simulink model "r2_b8a4x128f_4gbe"  (R2012b)
settings: Solver=VariableStepDiscrete  SolverMode=SingleTasking  StartTime=0.0  StopTime=1  RelTol=1e-3
undefined symbols (not defined in the file): fft_stages, n_ants, n_bits_xengs
libraries: xbsIndex_r4 x21845, casper_library_misc x157, xbsReplacements_r4 x24, casper_library_communications x8, casper_library_delays x8, xps_library x5
(part 77 of 182)

== system r2_b8a4x128f_4gbe/sys2/bf/fbf ==
  note: beam filtering
  note: requanitse
  note: accumulate
  note: create visibilities
  note: combine data from different antennas into beams
  note: beam steering
  note: antenna beam weights
  note: split polarisations and
      | duplicate for multiple beams
  note: TODO
  note: TODO
  note: control interface
  note: TODO
  synci : Inport
  di : Inport  Port=2
  deni : Inport  Port=3
  badi : Inport  Port=4
  timei : Inport  Port=5
  misci : Inport  Port=6
  ld_antenna : Inport  Port=7
  ld_stream : Inport  Port=8
  ld_wr_en : Inport  Port=9
  Assert : xbsIndex_r4/Assert  assert_type=on  type_source=Explicitly  gui_display_data_type=Boolean  arith_type=Boolean  n_bits=16  bin_pt=14  preci_type=Single  exp_width=8  frac_width=24  assert_rate=off  rate_source=Explicitly  period=1  output_port=on  block_type=assert
  Assert1 : xbsIndex_r4/Assert  assert_type=on  type_source=Explicitly  gui_display_data_type=Boolean  arith_type=Boolean  n_bits=16  bin_pt=14  preci_type=Single  exp_width=8  frac_width=24  assert_rate=off  rate_source=Explicitly  period=1  output_port=on  block_type=assert
  Assert2 : xbsIndex_r4/Assert  assert_type=on  type_source=Explicitly  gui_display_data_type=Boolean  arith_type=Boolean  n_bits=16  bin_pt=14  preci_type=Single  exp_width=8  frac_width=24  assert_rate=off  rate_source=Explicitly  period=1  output_port=on  block_type=assert
  Assert3 : xbsIndex_r4/Assert  assert_type=on  type_source=Explicitly  gui_display_data_type=Fixed-point  arith_type=Unsigned  n_bits=n_bits_in*2*2^polarisation_bits  bin_pt=0  preci_type=Single  exp_width=8  frac_width=24  assert_rate=off  rate_source=Explicitly  period=1  output_port=on  block_type=assert
  Assert4 : xbsIndex_r4/Assert  assert_type=on  type_source=Explicitly  gui_display_data_type=Fixed-point  arith_type=Unsigned  n_bits=timestamp_bits  bin_pt=0  preci_type=Single  exp_width=8  frac_width=24  assert_rate=off  rate_source=Explicitly  period=1  output_port=on  block_type=assert
  Assert6 : xbsIndex_r4/Assert  assert_type=on  type_source=Explicitly  gui_display_data_type=Fixed-point  arith_type=Unsigned  n_bits=ant_bits  bin_pt=0  preci_type=Single  exp_width=8  frac_width=24  assert_rate=off  rate_source=Explicitly  period=1  output_port=on  block_type=assert
  Assert7 : xbsIndex_r4/Assert  assert_type=on  type_source=Explicitly  gui_display_data_type=Fixed-point  arith_type=Unsigned  n_bits=polarisation_bits+beam_bits  bin_pt=0  preci_type=Single  exp_width=8  frac_width=24  assert_rate=off  rate_source=Explicitly  period=1  output_port=on  block_type=assert
  Assert9 : xbsIndex_r4/Assert  assert_type=on  type_source=Explicitly  gui_display_data_type=Boolean  arith_type=Boolean  n_bits=8  bin_pt=0  preci_type=Single  exp_width=8  frac_width=24  assert_rate=off  rate_source=Explicitly  period=1  output_port=on  block_type=assert
  Concat : xbsIndex_r4/Concat  num_inputs=2  dbl_ovrd=off  block_type=concat
  Concat1 : xbsIndex_r4/Concat  num_inputs=3  dbl_ovrd=off  block_type=concat
  Concat2 : xbsIndex_r4/Concat  num_inputs=2  dbl_ovrd=off  block_type=concat
  Concat3 : xbsIndex_r4/Concat  num_inputs=2  dbl_ovrd=off  block_type=concat
  Constant4 : xbsIndex_r4/Constant  const=0  gui_display_data_type=Fixed-point  arith_type=Unsigned  n_bits=freq_bits-beng_bits  bin_pt=0  preci_type=Single  exp_width=8  frac_width=24  explicit_period=on  period=1  equ=P=C  opselect=C  inp2=PCIN>>17  opr=+  inp1=P  carry=CIN  dbl_ovrd=off  block_type=constant
      settings: block_version=11.4
  Convert4 : xbsIndex_r4/Convert  gui_display_data_type=Fixed-point  arith_type=Unsigned  n_bits=1  bin_pt=0  float_type=Single  exp_bits=8  fraction_bits=24  quantization=Truncate  overflow=Wrap  en=off  latency=0  dbl_ovrd=off  pipeline=off  block_type=convert
  Delay{1..3,7} (4 alike) : xbsIndex_r4/Delay  rst=off  infoeditControl=Selection of Reset will increase slice count due to use of real FFs and instead of SRLs  en=off  latency=1  dbl_ovrd=off  reg_retiming=on  block_type=delay
  Gateway Out{,1..18} (19 alike) : xbsIndex_r4/Gateway Out  inherit_from_input=off  hdl_port=off  timing_constraint=None  locs_specified=off  LOCs={}  UseAsDAC=off  DACChannel='1'  block_type=gatewayout
      settings: infoedit="Gateway out block.  Converts Xilinx fixed point inputs into ouputs of type Simulink integer, double, or fixed point.<br><br>Hardware notes:  In hardware these blocks become top level output ports or are discarded, depending on how they are configured."  block_version=11.4
  Logical{,1..3} (4 alike) : xbsIndex_r4/Logical  logical_function=AND  inputs=2  en=off  latency=1  precision=Full  arith_type=Unsigned  n_bits=16  bin_pt=0  align_bp=on  dbl_ovrd=off  block_type=logical
  Reinterpret : xbsIndex_r4/Reinterpret  force_arith_type=on  arith_type="Signed  (2's comp)"  force_bin_pt=on  bin_pt=bin_pt_norm  block_type=reinterpret
      settings: infoedit="Changes signal type without altering the binary representation.   You can changed the signal between signed and unsigned, and relocate the binary point.<br><br>Hardware notes: In hardware this block costs nothing.<br><br>Example:  Suppose the input is 6 bits wide, signed, with 2 fractional bits, and the output is forced to unsigned with 0 fractional bits.  Then an input of -2.0 (1110.00 in binary 2's complement) becomes an output of 56 (111000 in binary)."
  Reinterpret1 : xbsIndex_r4/Reinterpret  force_arith_type=on  arith_type="Signed  (2's comp)"  force_bin_pt=on  bin_pt=bin_pt_norm  block_type=reinterpret
      settings: infoedit="Changes signal type without altering the binary representation.   You can changed the signal between signed and unsigned, and relocate the binary point.<br><br>Hardware notes: In hardware this block costs nothing.<br><br>Example:  Suppose the input is 6 bits wide, signed, with 2 fractional bits, and the output is forced to unsigned with 0 fractional bits.  Then an input of -2.0 (1110.00 in binary 2's complement) becomes an output of 56 (111000 in binary)."
  Reinterpret10 : xbsIndex_r4/Reinterpret  force_arith_type=on  arith_type=Unsigned  force_bin_pt=on  bin_pt=0  block_type=reinterpret
  Reinterpret11 : xbsIndex_r4/Reinterpret  force_arith_type=on  arith_type=Unsigned  force_bin_pt=on  bin_pt=0  block_type=reinterpret
  Reinterpret{2..3,6..9} (6 alike) : xbsIndex_r4/Reinterpret  force_arith_type=on  arith_type="Signed  (2's comp)"  force_bin_pt=on  bin_pt=0  block_type=reinterpret
      settings: infoedit="Changes signal type without altering the binary representation.   You can changed the signal between signed and unsigned, and relocate the binary point.<br><br>Hardware notes: In hardware this block costs nothing.<br><br>Example:  Suppose the input is 6 bits wide, signed, with 2 fractional bits, and the output is forced to unsigned with 0 fractional bits.  Then an input of -2.0 (1110.00 in binary 2's complement) becomes an output of 56 (111000 in binary)."
  Reinterpret4 : xbsIndex_r4/Reinterpret  force_arith_type=on  arith_type="Signed  (2's comp)"  force_bin_pt=on  bin_pt=bin_pt_out  block_type=reinterpret
      settings: infoedit="Changes signal type without altering the binary representation.   You can changed the signal between signed and unsigned, and relocate the binary point.<br><br>Hardware notes: In hardware this block costs nothing.<br><br>Example:  Suppose the input is 6 bits wide, signed, with 2 fractional bits, and the output is forced to unsigned with 0 fractional bits.  Then an input of -2.0 (1110.00 in binary 2's complement) becomes an output of 56 (111000 in binary)."
  Reinterpret5 : xbsIndex_r4/Reinterpret  force_arith_type=on  arith_type="Signed  (2's comp)"  force_bin_pt=on  bin_pt=bin_pt_out  block_type=reinterpret
      settings: infoedit="Changes signal type without altering the binary representation.   You can changed the signal between signed and unsigned, and relocate the binary point.<br><br>Hardware notes: In hardware this block costs nothing.<br><br>Example:  Suppose the input is 6 bits wide, signed, with 2 fractional bits, and the output is forced to unsigned with 0 fractional bits.  Then an input of -2.0 (1110.00 in binary 2's complement) becomes an output of 56 (111000 in binary)."
  Scope : Scope  NumInputPorts=5
      settings: YMin=0~-15~-15~0~10  YMax=1~12.5~12.5~1~11  SaveName=ScopeData2
  Scope1 : Scope  NumInputPorts=4
      settings: YMin=0~-1~0~-5  YMax=1~1~1~5  SaveName=ScopeData5
  Scope2 : Scope  NumInputPorts=4
      settings: YMin=0.1~-1~0~-5  YMax=1~0.5~1~5  SaveName=ScopeData14
  Scope3 : Scope  NumInputPorts=6
      settings: YMin=-1~3~3~3~3~-1  YMax=1~5~5~5~5~1  SaveName=ScopeData8
  Slice : xbsIndex_r4/Slice  nbits=n_bits_combine  boolean_output=off  mode=Lower Bit Location + Width  bit1=0  base1=MSB of Input  bit0=0  base0=LSB of Input  dbl_ovrd=off  block_type=slice
  Slice1 : xbsIndex_r4/Slice  nbits=n_bits_combine  boolean_output=off  mode=Lower Bit Location + Width  bit1=0  base1=MSB of Input  bit0=n_bits_combine  base0=LSB of Input  dbl_ovrd=off  block_type=slice
  Slice2 : xbsIndex_r4/Slice  nbits=n_bits_out  boolean_output=off  mode=Lower Bit Location + Width  bit1=0  base1=MSB of Input  bit0=0  base0=LSB of Input  dbl_ovrd=off  block_type=slice
  Slice3 : xbsIndex_r4/Slice  nbits=n_bits_out  boolean_output=off  mode=Lower Bit Location + Width  bit1=0  base1=MSB of Input  bit0=n_bits_out  base0=LSB of Input  dbl_ovrd=off  block_type=slice
  Slice4 : xbsIndex_r4/Slice  nbits=n_bits_out  boolean_output=off  mode=Lower Bit Location + Width  bit1=0  base1=MSB of Input  bit0=0  base0=LSB of Input  dbl_ovrd=off  block_type=slice
  Slice5 : xbsIndex_r4/Slice  nbits=n_bits_out  boolean_output=off  mode=Lower Bit Location + Width  bit1=0  base1=MSB of Input  bit0=n_bits_out  base0=LSB of Input  dbl_ovrd=off  block_type=slice
  Slice7 : xbsIndex_r4/Slice  nbits=1  boolean_output=on  mode=Lower Bit Location + Width  bit1=0  base1=MSB of Input  bit0=0  base0=LSB of Input  dbl_ovrd=off  block_type=slice
  apply_beam_weights : Subsystem  mask{vec_bits=ant_bits, stream_bits=polarisation_bits+beam_bits, stack_bits=(freq_bits-beng_bits)+stack_bits, type_in=1, n_bits_in=n_bits_in, bin_pt_in=bin_pt_in, complex_in=on, type_coeff=1, n_bits_coeff=n_bits_norm, bin_pt_coeff=bin_pt_norm, complex_coeff=off, mult_latency=mult_latency, n_bits_out=n_bits_in+n_bits_norm+1, bin_pt_out=bin_pt_in+bin_pt_norm, type_out=1, quantization=0, overflow=0, init_val=1}
      mask prompts: vec_bits "vector length (2^?)"; stream_bits "streams (2^?)"; stack_bits "stack factor (2^?)"; type_in "input type (Unsigned=0, Signed=1)"; n_bits_in "bit width in"; bin_pt_in "binary point in"; complex_in "complex input"; type_coeff "coefficient type (Unsigned=0, Signed=1)"; n_bits_coeff "coefficient bit width"; bin_pt_coeff "coefficient binary point"; complex_coeff "complex coefficients"; mult_latency "multiplier latency"; n_bits_out "output bit width"; bin_pt_out "output binary point"; type_out "output type (Unsigned=0, Signed=1)"; quantization "quantization strategy (Truncate=0, Round  (unbiased: +/- Inf)=1)"; overflow "overflow strategy (Wrap=0, Saturate=1, Flag as error=2)"; init_val "initial value"
      mask init: same as r2_b8a4x128f_4gbe/sys0/bf/fbf/apply_beam_weights
  bad_slc : xbsIndex_r4/Slice  nbits=1  boolean_output=on  mode=Upper Bit Location + Width  bit1=0  base1=MSB of Input  bit0=0  base0=LSB of Input  dbl_ovrd=off  block_type=slice
  bus_expand : Subsystem  AncestorBlock=casper_library_flow_control/bus_expand  mask(bus_expand){mode=divisions of equal size, outputNum=4, outputWidth=4, outputBinaryPt=3, outputArithmeticType=1, show_format=off, outputToWorkspace=off, variablePrefix=out, outputToModelAsWell=on}
      mask prompts: outputNum "Number of outputs:"; outputWidth "Output width:"; outputBinaryPt "Output binary point position:"; outputArithmeticType "Output arithmetic type (ufix=0, fix=1, bool=2):"; show_format "Print format string?"; outputToWorkspace "Output to workspace?"; variablePrefix "Variable name prefix:"; outputToModelAsWell "Output to model as well?"
      mask help:
      | Expands a 'bus' made using a bus_create or Xilinx
      | concat block.
      | The input will be divided into the specified number
      | of outputs with the specified arithmetic types.
      | Divisions are made from most significant bit.
      mask init: same as r2_b8a4x128f_4gbe/bus_expand
      settings: AttributesFormatString=4 outputs
      mask TypeOptions mode: divisions of equal size | divisions of arbitrary size
      mask Callback mode: bus_expand_callback();
      mask Callback outputWidth: bus_expand_callback();
      mask Callback outputToWorkspace: bus_expand_callback();
  combine : Subsystem  mask{freq_bits=freq_bits-beng_bits, ant_bits=ant_bits, stack_bits=stack_bits, stream_bits=beam_bits+polarisation_bits, n_bits_in=n_bits_in+n_bits_norm+1, bin_pt_in=bin_pt_in+bin_pt_norm, timestamp_bits=timestamp_bits, n_bits_accum=n_bits_combine, bram_latency=bram_latency, add_latency=add_latency}
      mask prompts: freq_bits "frequencies (2^?)"; ant_bits "antennas (2^?)"; stack_bits "stacking factor (2^?)"; stream_bits "input streams (2^?)"; n_bits_in "data bits in"; bin_pt_in "binary point in"; timestamp_bits "timestamp bits"; n_bits_accum "accumulator bits"; bram_latency "bram latency"; add_latency "add latency"
  duplicate : Subsystem  mask{ant_bits=ant_bits, freq_bits=freq_bits-beng_bits, stack_bits=stack_bits, beam_bits=beam_bits, polarisation_bits=polarisation_bits, n_bits_in=n_bits_in}
      mask prompts: ant_bits "antennas (2^?)"; freq_bits "frequencies (2^?)"; stack_bits "stacking factor (2^?)"; beam_bits "beams (2^?)"; polarisation_bits "polarisations (2^?)"; n_bits_in "data bits in"
      mask init:
      | set_param([gcb,'/beam_replicate'], ...
      |     'replication', '2^beam_bits');
      | set_param([gcb,'/pol_replicate'], ...
      |     'replication', '2^polarisation_bits');
  filter : Subsystem  mask{stream_bits=beam_bits+polarisation_bits, vec_bits=freq_bits-beng_bits, stack_bits=stack_bits, output_enabled=off}
      mask prompts: stream_bits "streams (2^?)"; vec_bits "vector length (2^?)"; stack_bits "stack factor (2^?)"; output_enabled "output enabled by default?"
      mask init: same as r2_b8a4x128f_4gbe/sys0/bf/fbf/filter
  ld_freq5 : xbsIndex_r4/Slice  nbits=1  boolean_output=off  mode=Two Bit Locations  bit1=-(timestamp_bits+1)  base1=MSB of Input  bit0=0  base0=LSB of Input  dbl_ovrd=off  block_type=slice
  misco_slc : xbsIndex_r4/Slice  nbits=1  boolean_output=off  mode=Two Bit Locations  bit1=-timestamp_bits  base1=MSB of Input  bit0=0  base0=LSB of Input  dbl_ovrd=off  block_type=slice
  pipeline1 : Subsystem  AncestorBlock=casper_library_delays/pipeline  mask(pipeline){latency=2}
      mask help:
      | An explicitly laid-out delay line to avoid mapping to SRL16s
      | for use in pipelining to help achieve timing closure.
      mask init:
      | pipeline_init(gcb,'latency',latency);
      settings: AttributesFormatString=Latency = %<latency>
      mask Display:
      | port_label('input', 1, 'd');
      | port_label('output', 1, 'q');
      | disp(['Z^-', num2str(latency)]);
  pipeline10 : Subsystem  AncestorBlock=casper_library_delays/pipeline  mask(pipeline){latency=2}
      mask help:
      | An explicitly laid-out delay line to avoid mapping to SRL16s
      | for use in pipelining to help achieve timing closure.
      mask init:
      | pipeline_init(gcb,'latency',latency);
      settings: AttributesFormatString=Latency = %<latency>
      mask Display:
      | port_label('input', 1, 'd');
      | port_label('output', 1, 'q');
      | disp(['Z^-', num2str(latency)]);
  pipeline11 : Subsystem  AncestorBlock=casper_library_delays/pipeline  mask(pipeline){latency=2}
      mask help:
      | An explicitly laid-out delay line to avoid mapping to SRL16s
      | for use in pipelining to help achieve timing closure.
      mask init:
      | pipeline_init(gcb,'latency',latency);
      settings: AttributesFormatString=Latency = %<latency>
      mask Display:
      | port_label('input', 1, 'd');
      | port_label('output', 1, 'q');
      | disp(['Z^-', num2str(latency)]);
  pipeline12 : Subsystem  AncestorBlock=casper_library_delays/pipeline  mask(pipeline){latency=2}
      mask help:
      | An explicitly laid-out delay line to avoid mapping to SRL16s
      | for use in pipelining to help achieve timing closure.
      mask init:
      | pipeline_init(gcb,'latency',latency);
      settings: AttributesFormatString=Latency = %<latency>
      mask Display:
      | port_label('input', 1, 'd');
      | port_label('output', 1, 'q');
      | disp(['Z^-', num2str(latency)]);
  pipeline13 : Subsystem  AncestorBlock=casper_library_delays/pipeline  mask(pipeline){latency=2}
      mask help:
      | An explicitly laid-out delay line to avoid mapping to SRL16s
      | for use in pipelining to help achieve timing closure.
      mask init:
      | pipeline_init(gcb,'latency',latency);
      settings: AttributesFormatString=Latency = %<latency>
      mask Display:
      | port_label('input', 1, 'd');
      | port_label('output', 1, 'q');
      | disp(['Z^-', num2str(latency)]);
  pipeline14 : Subsystem  AncestorBlock=casper_library_delays/pipeline  mask(pipeline){latency=2}
      mask help:
      | An explicitly laid-out delay line to avoid mapping to SRL16s
      | for use in pipelining to help achieve timing closure.
      mask init:
      | pipeline_init(gcb,'latency',latency);
      settings: AttributesFormatString=Latency = %<latency>
      mask Display:
      | port_label('input', 1, 'd');
      | port_label('output', 1, 'q');
      | disp(['Z^-', num2str(latency)]);
  pipeline15 : Subsystem  AncestorBlock=casper_library_delays/pipeline  mask(pipeline){latency=2}
      mask help:
      | An explicitly laid-out delay line to avoid mapping to SRL16s
      | for use in pipelining to help achieve timing closure.
      mask init:
      | pipeline_init(gcb,'latency',latency);
      settings: AttributesFormatString=Latency = %<latency>
      mask Display:
      | port_label('input', 1, 'd');
      | port_label('output', 1, 'q');
      | disp(['Z^-', num2str(latency)]);
  pipeline16 : Subsystem  AncestorBlock=casper_library_delays/pipeline  mask(pipeline){latency=2}
      mask help:
      | An explicitly laid-out delay line to avoid mapping to SRL16s
      | for use in pipelining to help achieve timing closure.
      mask init:
      | pipeline_init(gcb,'latency',latency);
      settings: AttributesFormatString=Latency = %<latency>
      mask Display:
      | port_label('input', 1, 'd');
      | port_label('output', 1, 'q');
      | disp(['Z^-', num2str(latency)]);
  pipeline2 : Subsystem  AncestorBlock=casper_library_delays/pipeline  mask(pipeline){latency=2}
      mask help:
      | An explicitly laid-out delay line to avoid mapping to SRL16s
      | for use in pipelining to help achieve timing closure.
      mask init:
      | pipeline_init(gcb,'latency',latency);
      settings: AttributesFormatString=Latency = %<latency>
      mask Display:
      | port_label('input', 1, 'd');
      | port_label('output', 1, 'q');
      | disp(['Z^-', num2str(latency)]);
  pipeline3 : Subsystem  AncestorBlock=casper_library_delays/pipeline  mask(pipeline){latency=2}
      mask help:
      | An explicitly laid-out delay line to avoid mapping to SRL16s
      | for use in pipelining to help achieve timing closure.
      mask init:
      | pipeline_init(gcb,'latency',latency);
      settings: AttributesFormatString=Latency = %<latency>
      mask Display:
      | port_label('input', 1, 'd');
      | port_label('output', 1, 'q');
      | disp(['Z^-', num2str(latency)]);
  pipeline4 : Subsystem  AncestorBlock=casper_library_delays/pipeline  mask(pipeline){latency=2}
      mask help:
      | An explicitly laid-out delay line to avoid mapping to SRL16s
      | for use in pipelining to help achieve timing closure.
      mask init:
      | pipeline_init(gcb,'latency',latency);
      settings: AttributesFormatString=Latency = %<latency>
      mask Display:
      | port_label('input', 1, 'd');
      | port_label('output', 1, 'q');
      | disp(['Z^-', num2str(latency)]);
  pipeline5 : Subsystem  AncestorBlock=casper_library_delays/pipeline  mask(pipeline){latency=2}
      mask help:
      | An explicitly laid-out delay line to avoid mapping to SRL16s
      | for use in pipelining to help achieve timing closure.
      mask init:
      | pipeline_init(gcb,'latency',latency);
      settings: AttributesFormatString=Latency = %<latency>
      mask Display:
      | port_label('input', 1, 'd');
      | port_label('output', 1, 'q');
      | disp(['Z^-', num2str(latency)]);
  pipeline6 : Subsystem  AncestorBlock=casper_library_delays/pipeline  mask(pipeline){latency=2}
      mask help:
      | An explicitly laid-out delay line to avoid mapping to SRL16s
      | for use in pipelining to help achieve timing closure.
      mask init:
      | pipeline_init(gcb,'latency',latency);
      settings: AttributesFormatString=Latency = %<latency>
      mask Display:
      | port_label('input', 1, 'd');
      | port_label('output', 1, 'q');
      | disp(['Z^-', num2str(latency)]);
  pipeline7 : Subsystem  AncestorBlock=casper_library_delays/pipeline  mask(pipeline){latency=2}
      mask help:
      | An explicitly laid-out delay line to avoid mapping to SRL16s
      | for use in pipelining to help achieve timing closure.
      mask init:
      | pipeline_init(gcb,'latency',latency);
      settings: AttributesFormatString=Latency = %<latency>
      mask Display:
      | port_label('input', 1, 'd');
      | port_label('output', 1, 'q');
      | disp(['Z^-', num2str(latency)]);
  pipeline8 : Subsystem  AncestorBlock=casper_library_delays/pipeline  mask(pipeline){latency=2}
      mask help:
      | An explicitly laid-out delay line to avoid mapping to SRL16s
      | for use in pipelining to help achieve timing closure.
      mask init:
      | pipeline_init(gcb,'latency',latency);
      settings: AttributesFormatString=Latency = %<latency>
      mask Display:
      | port_label('input', 1, 'd');
      | port_label('output', 1, 'q');
      | disp(['Z^-', num2str(latency)]);
  pipeline9 : Subsystem  AncestorBlock=casper_library_delays/pipeline  mask(pipeline){latency=2}
      mask help:
      | An explicitly laid-out delay line to avoid mapping to SRL16s
      | for use in pipelining to help achieve timing closure.
      mask init:
      | pipeline_init(gcb,'latency',latency);
      settings: AttributesFormatString=Latency = %<latency>
      mask Display:
      | port_label('input', 1, 'd');
      | port_label('output', 1, 'q');
      | disp(['Z^-', num2str(latency)]);
  requantise : Subsystem  mask{vec_bits=freq_bits-beng_bits, stream_bits=polarisation_bits+beam_bits, stack_bits=stack_bits, type_in=1, n_bits_in=n_bits_combine, bin_pt_in=bin_pt_in+bin_pt_norm, complex_in=on, type_coeff=1, n_bits_coeff=n_bits_requant, bin_pt_coeff=bin_pt_requant, complex_coeff=off, mult_latency=mult_latency, conv_latency=conv_latency, n_bits_out=n_bits_out, bin_pt_out=bin_pt_out, type_out=1, quantization=1, overflow=1, init_val=1}
      mask prompts: vec_bits "vector length (2^?)"; stream_bits "streams (2^?)"; stack_bits "stack factor (2^?)"; type_in "input type (Unsigned=0, Signed=1)"; n_bits_in "bit width in"; bin_pt_in "binary point in"; complex_in "complex input"; type_coeff "coefficient type (Unsigned=0, Signed=1)"; n_bits_coeff "coefficient bit width"; bin_pt_coeff "coefficient binary point"; complex_coeff "complex coefficients"; mult_latency "multiplier latency"; conv_latency "convert latency"; n_bits_out "output bit width"; bin_pt_out "output binary point"; type_out "output type (Unsigned=0, Signed=1)"; quantization "quantization strategy (Truncate=0, Round  (unbiased: +/- Inf)=1)"; overflow "overflow strategy (Wrap=0, Saturate=1, Flag as error=2)"; init_val "initial value"
      mask init: same as r2_b8a4x128f_4gbe/sys0/bf/fbf/requantise
  sync_gen : Subsystem
  time_slc : xbsIndex_r4/Slice  nbits=timestamp_bits  boolean_output=off  mode=Upper Bit Location + Width  bit1=-1  base1=MSB of Input  bit0=0  base0=LSB of Input  dbl_ovrd=off  block_type=slice
  timeo_slc : xbsIndex_r4/Slice  nbits=timestamp_bits  boolean_output=off  mode=Upper Bit Location + Width  bit1=0  base1=MSB of Input  bit0=0  base0=LSB of Input  dbl_ovrd=off  block_type=slice
  synco : Outport
  do : Outport  Port=2
  deno : Outport  Port=3
  timeo : Outport  Port=4
  misco : Outport  Port=5
  bw_value_out : Outport  Port=6
  quant_value_out : Outport  Port=7
  filter_value_out : Outport  Port=8
  wires:
  sync_gen/3(do) -> duplicate/3(di)
  sync_gen/6(misco) -> duplicate/6(misci)
  sync_gen/5(timeo) -> duplicate/5(timei)
  sync_gen/2(dvalid) -> duplicate/2(eni)
  sync_gen/1(synco) -> duplicate/1(synci)
  sync_gen/4(bado) -> duplicate/4(badi)
  misci/1 -> sync_gen/6(misci)
  Assert4/1 -> sync_gen/5(timei)
  Assert2/1 -> sync_gen/4(badi)
  Assert3/1 -> sync_gen/3(di)
  Assert/1 -> sync_gen/1(synci)
  Assert1/1 -> sync_gen/2(en)
  Assert9/1 -> [control_en]
  ld_wr_en/1 -> Assert9/1
  Assert7/1 -> [stream]
  ld_stream/1 -> Assert7/1
  Assert6/1 -> [antenna]
  ld_antenna/1 -> Assert6/1
  Gateway Out5/1 -> Scope1/4
  Gateway Out4/1 -> Scope1/3
  Gateway Out3/1 -> Scope1/2
  Gateway Out18/1 -> Scope1/1
  [requantise_synco] -> Gateway Out18/1
  filter/1(synco) -> [filter_synco], synco/1
  requantise/1(synco) -> pipeline4/1(d), [requantise_synco]
  [requantise_val_out] -> quant_value_out/1
  [filter_val_out] -> filter_value_out/1
  requantise/5(valo) -> [requantise_val_out]
  filter/5(valo) -> [filter_val_out]
  [bw_val_out] -> bw_value_out/1
  apply_beam_weights/5(valo) -> [bw_val_out]
  apply_beam_weights/4(misco) -> pipeline11/1(d)
  [filter_synco] -> Gateway Out17/1
  Gateway Out9/1 -> Scope2/4
  Gateway Out8/1 -> Scope2/3
  Gateway Out7/1 -> Scope2/2
  Gateway Out17/1 -> Scope2/1
  Gateway Out14/1 -> Scope3/6
  Gateway Out13/1 -> Scope3/5
  Gateway Out12/1 -> Scope3/4
  Gateway Out11/1 -> Scope3/3
  Gateway Out10/1 -> Scope3/2
  Gateway Out16/1 -> Scope3/1
  [gen_sync] -> Gateway Out16/1
  Gateway Out6/1 -> Scope/5
  Gateway Out2/1 -> Scope/4
  Gateway Out1/1 -> Scope/3
  Gateway Out/1 -> Scope/2
  Gateway Out15/1 -> Scope/1
  [combine_sync] -> Gateway Out15/1
  filter/3(eno) -> [filter_eno], deno/1
  filter/2(do) -> [filter_dout], do/1
  requantise/4(misco) -> pipeline7/1(d)
  requantise/3(eno) -> pipeline6/1(d), [requantise_eno]
  requantise/2(dout) -> pipeline5/1(d), [requantise_dout]
  combine/1(synco) -> pipeline15/1(d), [combine_sync]
  apply_beam_weights/1(synco) -> pipeline8/1(d)
  filter/4(misco) -> misco_slc/1, timeo_slc/1
  [gen_do] -> bus_expand/1(bus_in)
  bus_expand/4(lsb_out1) -> Reinterpret9/1
  bus_expand/3(out2) -> Reinterpret8/1
  [gen_eno] -> Gateway Out14/1
  Reinterpret9/1 -> Gateway Out13/1
  Reinterpret8/1 -> Gateway Out12/1
  Reinterpret7/1 -> Gateway Out11/1
  Reinterpret6/1 -> Gateway Out10/1
  bus_expand/2(out3) -> Reinterpret7/1
  bus_expand/1(msb_out4) -> Reinterpret6/1
  Convert4/1 -> Slice7/1
  [bf_value_dupl] -> Delay3/1
  Reinterpret5/1 -> Gateway Out8/1
  Reinterpret4/1 -> Gateway Out7/1
  [filter_eno] -> Gateway Out9/1
  [filter_dout] -> Slice4/1, Slice5/1
  Slice4/1 -> Reinterpret5/1
  Slice5/1 -> Reinterpret4/1
  [stream] -> filter/5(stream)
  [combine_time] -> Gateway Out6/1
  Concat3/1 -> pipeline3/1(d)
  combine/5(misco) -> Concat3/2
  combine/4(timeo) -> [combine_time], Concat3/1
  time_slc/1 -> combine/5(timei)
  duplicate/5(timeo) -> Concat1/2
  duplicate/4(bado) -> Concat1/1
  duplicate/3(eno) -> pipeline14/1(d), [gen_eno]
  misco_slc/1 -> misco/1
  timeo_slc/1 -> timeo/1
  Reinterpret3/1 -> Gateway Out4/1
  Reinterpret2/1 -> Gateway Out3/1
  [requantise_eno] -> Gateway Out5/1
  [requantise_dout] -> Slice3/1, Slice2/1
  Slice2/1 -> Reinterpret3/1
  Slice3/1 -> Reinterpret2/1
  Reinterpret1/1 -> Gateway Out1/1
  Reinterpret/1 -> Gateway Out/1
  [combine_eno] -> Gateway Out2/1
  [combine_sum] -> Slice/1, Slice1/1
  Slice/1 -> Reinterpret1/1
  Slice1/1 -> Reinterpret/1
  apply_beam_weights/3(eno) -> pipeline10/1(d)
  apply_beam_weights/2(dout) -> pipeline9/1(d)
  combine/3(eno) -> pipeline2/1(d), [combine_eno]
  combine/2(sum) -> pipeline1/1(d), [combine_sum]
  Delay7/1 -> Reinterpret11/1
  duplicate/6(misco) -> Concat1/3
  Logical1/1 -> apply_beam_weights/7(we)
  Delay2/1 -> Reinterpret10/1
  Concat/1 -> apply_beam_weights/5(index)
  timei/1 -> Assert4/1
  ld_freq5/1 -> combine/6(misci)
  bad_slc/1 -> combine/4(bad)
  Concat1/1 -> pipeline16/1(d)
  duplicate/2(do) -> pipeline13/1(d), [gen_do]
  duplicate/1(synco) -> pipeline12/1(d), [gen_sync]
  badi/1 -> Assert2/1
  di/1 -> Assert3/1
  deni/1 -> Assert1/1
  synci/1 -> Assert/1
  [antenna] -> Concat/1
  [stream] -> Concat/2
  [frequency] -> Concat2/1
  [stream] -> Concat2/2
  Concat2/1 -> requantise/5(index)
  Constant4/1 -> [frequency]
  Delay1/1 -> filter/6(vali)
  Slice7/1 -> duplicate/8(sim_type)
  Reinterpret10/1 -> apply_beam_weights/6(vali)
  Reinterpret11/1 -> requantise/6(vali)
  Delay3/1 -> Convert4/1
  [bf_value_filt] -> Delay1/1
  [bf_value_bw] -> Delay2/1
  [bf_value_quant] -> Delay7/1
  Logical2/1 -> requantise/7(we)
  Logical3/1 -> filter/7(ld)
  [control_en] -> Logical/2
  [bf_valctrl_dupl] -> Logical/1
  Logical/1 -> duplicate/7(sim_ld)
  [control_en] -> Logical1/2
  [bf_valctrl_bw] -> Logical1/1
  [control_en] -> Logical2/2
  [bf_valctrl_quant] -> Logical2/1
  [control_en] -> Logical3/2
  [bf_valctrl_filt] -> Logical3/1
  pipeline4/1(q) -> filter/1(synci)
  pipeline5/1(q) -> filter/2(di)
  pipeline6/1(q) -> filter/3(eni)
  pipeline7/1(q) -> filter/4(misci)
  pipeline15/1(q) -> requantise/1(synci)
  pipeline1/1(q) -> requantise/2(din)
  pipeline2/1(q) -> requantise/3(den)
  pipeline3/1(q) -> requantise/4(misci)
  pipeline8/1(q) -> combine/1(synci)
  pipeline9/1(q) -> combine/2(data)
  pipeline10/1(q) -> combine/3(den)
  pipeline11/1(q) -> ld_freq5/1, time_slc/1, bad_slc/1
  pipeline12/1(q) -> apply_beam_weights/1(synci)
  pipeline13/1(q) -> apply_beam_weights/2(din)
  pipeline14/1(q) -> apply_beam_weights/3(den)
  pipeline16/1(q) -> apply_beam_weights/4(misci)

== system r2_b8a4x128f_4gbe/sys2/bus_relational/a_debus ==
  bus_in : Inport
  reinterpret{1..19} (19 alike) : xbsIndex_r4/Reinterpret  force_arith_type=on  arith_type=Unsigned  force_bin_pt=on  bin_pt=0  block_type=reinterpret
  slice1 : xbsIndex_r4/Slice  nbits=1  boolean_output=off  mode=Upper Bit Location + Width  bit1=-18  base1=MSB of Input  bit0=0  base0=LSB of Input  dbl_ovrd=off  block_type=slice
  slice10 : xbsIndex_r4/Slice  nbits=1  boolean_output=off  mode=Upper Bit Location + Width  bit1=-9  base1=MSB of Input  bit0=0  base0=LSB of Input  dbl_ovrd=off  block_type=slice
  slice11 : xbsIndex_r4/Slice  nbits=1  boolean_output=off  mode=Upper Bit Location + Width  bit1=-8  base1=MSB of Input  bit0=0  base0=LSB of Input  dbl_ovrd=off  block_type=slice
  slice12 : xbsIndex_r4/Slice  nbits=1  boolean_output=off  mode=Upper Bit Location + Width  bit1=-7  base1=MSB of Input  bit0=0  base0=LSB of Input  dbl_ovrd=off  block_type=slice
  slice13 : xbsIndex_r4/Slice  nbits=1  boolean_output=off  mode=Upper Bit Location + Width  bit1=-6  base1=MSB of Input  bit0=0  base0=LSB of Input  dbl_ovrd=off  block_type=slice
  slice14 : xbsIndex_r4/Slice  nbits=1  boolean_output=off  mode=Upper Bit Location + Width  bit1=-5  base1=MSB of Input  bit0=0  base0=LSB of Input  dbl_ovrd=off  block_type=slice
  slice15 : xbsIndex_r4/Slice  nbits=1  boolean_output=off  mode=Upper Bit Location + Width  bit1=-4  base1=MSB of Input  bit0=0  base0=LSB of Input  dbl_ovrd=off  block_type=slice
  slice16 : xbsIndex_r4/Slice  nbits=1  boolean_output=off  mode=Upper Bit Location + Width  bit1=-3  base1=MSB of Input  bit0=0  base0=LSB of Input  dbl_ovrd=off  block_type=slice
  slice17 : xbsIndex_r4/Slice  nbits=1  boolean_output=off  mode=Upper Bit Location + Width  bit1=-2  base1=MSB of Input  bit0=0  base0=LSB of Input  dbl_ovrd=off  block_type=slice
  slice18 : xbsIndex_r4/Slice  nbits=1  boolean_output=off  mode=Upper Bit Location + Width  bit1=-1  base1=MSB of Input  bit0=0  base0=LSB of Input  dbl_ovrd=off  block_type=slice
  slice19 : xbsIndex_r4/Slice  nbits=1  boolean_output=off  mode=Upper Bit Location + Width  bit1=0  base1=MSB of Input  bit0=0  base0=LSB of Input  dbl_ovrd=off  block_type=slice
  slice2 : xbsIndex_r4/Slice  nbits=1  boolean_output=off  mode=Upper Bit Location + Width  bit1=-17  base1=MSB of Input  bit0=0  base0=LSB of Input  dbl_ovrd=off  block_type=slice
  slice3 : xbsIndex_r4/Slice  nbits=1  boolean_output=off  mode=Upper Bit Location + Width  bit1=-16  base1=MSB of Input  bit0=0  base0=LSB of Input  dbl_ovrd=off  block_type=slice
  slice4 : xbsIndex_r4/Slice  nbits=1  boolean_output=off  mode=Upper Bit Location + Width  bit1=-15  base1=MSB of Input  bit0=0  base0=LSB of Input  dbl_ovrd=off  block_type=slice
  slice5 : xbsIndex_r4/Slice  nbits=1  boolean_output=off  mode=Upper Bit Location + Width  bit1=-14  base1=MSB of Input  bit0=0  base0=LSB of Input  dbl_ovrd=off  block_type=slice
  slice6 : xbsIndex_r4/Slice  nbits=1  boolean_output=off  mode=Upper Bit Location + Width  bit1=-13  base1=MSB of Input  bit0=0  base0=LSB of Input  dbl_ovrd=off  block_type=slice
  slice7 : xbsIndex_r4/Slice  nbits=1  boolean_output=off  mode=Upper Bit Location + Width  bit1=-12  base1=MSB of Input  bit0=0  base0=LSB of Input  dbl_ovrd=off  block_type=slice
  slice8 : xbsIndex_r4/Slice  nbits=1  boolean_output=off  mode=Upper Bit Location + Width  bit1=-11  base1=MSB of Input  bit0=0  base0=LSB of Input  dbl_ovrd=off  block_type=slice
  slice9 : xbsIndex_r4/Slice  nbits=1  boolean_output=off  mode=Upper Bit Location + Width  bit1=-10  base1=MSB of Input  bit0=0  base0=LSB of Input  dbl_ovrd=off  block_type=slice
  msb_out19 : Outport
  out18 : Outport  Port=2
  out17 : Outport  Port=3
  out16 : Outport  Port=4
  out15 : Outport  Port=5
  out14 : Outport  Port=6
  out13 : Outport  Port=7
  out12 : Outport  Port=8
  out11 : Outport  Port=9
  out10 : Outport  Port=10
  out9 : Outport  Port=11
  out8 : Outport  Port=12
  out7 : Outport  Port=13
  out6 : Outport  Port=14
  out5 : Outport  Port=15
  out4 : Outport  Port=16
  out3 : Outport  Port=17
  out2 : Outport  Port=18
  lsb_out1 : Outport  Port=19
  wires:
  bus_in/1 -> slice19/1, slice18/1, slice17/1, slice16/1, slice15/1, slice14/1, slice13/1, slice12/1, slice11/1, slice10/1, slice9/1, slice8/1, slice7/1, slice6/1, slice5/1, slice4/1, slice3/1, slice2/1, slice1/1
  slice19/1 -> reinterpret19/1
  reinterpret19/1 -> msb_out19/1
  slice18/1 -> reinterpret18/1
  reinterpret18/1 -> out18/1
  slice17/1 -> reinterpret17/1
  reinterpret17/1 -> out17/1
  slice16/1 -> reinterpret16/1
  reinterpret16/1 -> out16/1
  slice15/1 -> reinterpret15/1
  reinterpret15/1 -> out15/1
  slice14/1 -> reinterpret14/1
  reinterpret14/1 -> out14/1
  slice13/1 -> reinterpret13/1
  reinterpret13/1 -> out13/1
  slice12/1 -> reinterpret12/1
  reinterpret12/1 -> out12/1
  slice11/1 -> reinterpret11/1
  reinterpret11/1 -> out11/1
  slice10/1 -> reinterpret10/1
  reinterpret10/1 -> out10/1
  slice9/1 -> reinterpret9/1
  reinterpret9/1 -> out9/1
  slice8/1 -> reinterpret8/1
  reinterpret8/1 -> out8/1
  slice7/1 -> reinterpret7/1
  reinterpret7/1 -> out7/1
  slice6/1 -> reinterpret6/1
  reinterpret6/1 -> out6/1
  slice5/1 -> reinterpret5/1
  reinterpret5/1 -> out5/1
  slice4/1 -> reinterpret4/1
  reinterpret4/1 -> out4/1
  slice3/1 -> reinterpret3/1
  reinterpret3/1 -> out3/1
  slice2/1 -> reinterpret2/1
  reinterpret2/1 -> out2/1
  slice1/1 -> reinterpret1/1
  reinterpret1/1 -> lsb_out1/1

== system r2_b8a4x128f_4gbe/sys2/bus_relational/b_debus ==
  bus_in : Inport
  reinterpret{1..19} (19 alike) : xbsIndex_r4/Reinterpret  force_arith_type=on  arith_type=Unsigned  force_bin_pt=on  bin_pt=0  block_type=reinterpret
  slice1 : xbsIndex_r4/Slice  nbits=1  boolean_output=off  mode=Upper Bit Location + Width  bit1=-18  base1=MSB of Input  bit0=0  base0=LSB of Input  dbl_ovrd=off  block_type=slice
  slice10 : xbsIndex_r4/Slice  nbits=1  boolean_output=off  mode=Upper Bit Location + Width  bit1=-9  base1=MSB of Input  bit0=0  base0=LSB of Input  dbl_ovrd=off  block_type=slice
  slice11 : xbsIndex_r4/Slice  nbits=1  boolean_output=off  mode=Upper Bit Location + Width  bit1=-8  base1=MSB of Input  bit0=0  base0=LSB of Input  dbl_ovrd=off  block_type=slice
  slice12 : xbsIndex_r4/Slice  nbits=1  boolean_output=off  mode=Upper Bit Location + Width  bit1=-7  base1=MSB of Input  bit0=0  base0=LSB of Input  dbl_ovrd=off  block_type=slice
  slice13 : xbsIndex_r4/Slice  nbits=1  boolean_output=off  mode=Upper Bit Location + Width  bit1=-6  base1=MSB of Input  bit0=0  base0=LSB of Input  dbl_ovrd=off  block_type=slice
  slice14 : xbsIndex_r4/Slice  nbits=1  boolean_output=off  mode=Upper Bit Location + Width  bit1=-5  base1=MSB of Input  bit0=0  base0=LSB of Input  dbl_ovrd=off  block_type=slice
  slice15 : xbsIndex_r4/Slice  nbits=1  boolean_output=off  mode=Upper Bit Location + Width  bit1=-4  base1=MSB of Input  bit0=0  base0=LSB of Input  dbl_ovrd=off  block_type=slice
  slice16 : xbsIndex_r4/Slice  nbits=1  boolean_output=off  mode=Upper Bit Location + Width  bit1=-3  base1=MSB of Input  bit0=0  base0=LSB of Input  dbl_ovrd=off  block_type=slice
  slice17 : xbsIndex_r4/Slice  nbits=1  boolean_output=off  mode=Upper Bit Location + Width  bit1=-2  base1=MSB of Input  bit0=0  base0=LSB of Input  dbl_ovrd=off  block_type=slice
  slice18 : xbsIndex_r4/Slice  nbits=1  boolean_output=off  mode=Upper Bit Location + Width  bit1=-1  base1=MSB of Input  bit0=0  base0=LSB of Input  dbl_ovrd=off  block_type=slice
  slice19 : xbsIndex_r4/Slice  nbits=1  boolean_output=off  mode=Upper Bit Location + Width  bit1=0  base1=MSB of Input  bit0=0  base0=LSB of Input  dbl_ovrd=off  block_type=slice
  slice2 : xbsIndex_r4/Slice  nbits=1  boolean_output=off  mode=Upper Bit Location + Width  bit1=-17  base1=MSB of Input  bit0=0  base0=LSB of Input  dbl_ovrd=off  block_type=slice
  slice3 : xbsIndex_r4/Slice  nbits=1  boolean_output=off  mode=Upper Bit Location + Width  bit1=-16  base1=MSB of Input  bit0=0  base0=LSB of Input  dbl_ovrd=off  block_type=slice
  slice4 : xbsIndex_r4/Slice  nbits=1  boolean_output=off  mode=Upper Bit Location + Width  bit1=-15  base1=MSB of Input  bit0=0  base0=LSB of Input  dbl_ovrd=off  block_type=slice
  slice5 : xbsIndex_r4/Slice  nbits=1  boolean_output=off  mode=Upper Bit Location + Width  bit1=-14  base1=MSB of Input  bit0=0  base0=LSB of Input  dbl_ovrd=off  block_type=slice
  slice6 : xbsIndex_r4/Slice  nbits=1  boolean_output=off  mode=Upper Bit Location + Width  bit1=-13  base1=MSB of Input  bit0=0  base0=LSB of Input  dbl_ovrd=off  block_type=slice
  slice7 : xbsIndex_r4/Slice  nbits=1  boolean_output=off  mode=Upper Bit Location + Width  bit1=-12  base1=MSB of Input  bit0=0  base0=LSB of Input  dbl_ovrd=off  block_type=slice
  slice8 : xbsIndex_r4/Slice  nbits=1  boolean_output=off  mode=Upper Bit Location + Width  bit1=-11  base1=MSB of Input  bit0=0  base0=LSB of Input  dbl_ovrd=off  block_type=slice
  slice9 : xbsIndex_r4/Slice  nbits=1  boolean_output=off  mode=Upper Bit Location + Width  bit1=-10  base1=MSB of Input  bit0=0  base0=LSB of Input  dbl_ovrd=off  block_type=slice
  msb_out19 : Outport
  out18 : Outport  Port=2
  out17 : Outport  Port=3
  out16 : Outport  Port=4
  out15 : Outport  Port=5
  out14 : Outport  Port=6
  out13 : Outport  Port=7
  out12 : Outport  Port=8
  out11 : Outport  Port=9
  out10 : Outport  Port=10
  out9 : Outport  Port=11
  out8 : Outport  Port=12
  out7 : Outport  Port=13
  out6 : Outport  Port=14
  out5 : Outport  Port=15
  out4 : Outport  Port=16
  out3 : Outport  Port=17
  out2 : Outport  Port=18
  lsb_out1 : Outport  Port=19
  wires:
  bus_in/1 -> slice19/1, slice18/1, slice17/1, slice16/1, slice15/1, slice14/1, slice13/1, slice12/1, slice11/1, slice10/1, slice9/1, slice8/1, slice7/1, slice6/1, slice5/1, slice4/1, slice3/1, slice2/1, slice1/1
  slice19/1 -> reinterpret19/1
  reinterpret19/1 -> msb_out19/1
  slice18/1 -> reinterpret18/1
  reinterpret18/1 -> out18/1
  slice17/1 -> reinterpret17/1
  reinterpret17/1 -> out17/1
  slice16/1 -> reinterpret16/1
  reinterpret16/1 -> out16/1
  slice15/1 -> reinterpret15/1
  reinterpret15/1 -> out15/1
  slice14/1 -> reinterpret14/1
  reinterpret14/1 -> out14/1
  slice13/1 -> reinterpret13/1
  reinterpret13/1 -> out13/1
  slice12/1 -> reinterpret12/1
  reinterpret12/1 -> out12/1
  slice11/1 -> reinterpret11/1
  reinterpret11/1 -> out11/1
  slice10/1 -> reinterpret10/1
  reinterpret10/1 -> out10/1
  slice9/1 -> reinterpret9/1
  reinterpret9/1 -> out9/1
  slice8/1 -> reinterpret8/1
  reinterpret8/1 -> out8/1
  slice7/1 -> reinterpret7/1
  reinterpret7/1 -> out7/1
  slice6/1 -> reinterpret6/1
  reinterpret6/1 -> out6/1
  slice5/1 -> reinterpret5/1
  reinterpret5/1 -> out5/1
  slice4/1 -> reinterpret4/1
  reinterpret4/1 -> out4/1
  slice3/1 -> reinterpret3/1
  reinterpret3/1 -> out3/1
  slice2/1 -> reinterpret2/1
  reinterpret2/1 -> out2/1
  slice1/1 -> reinterpret1/1
  reinterpret1/1 -> lsb_out1/1

== system r2_b8a4x128f_4gbe/sys2/bus_relational/bussify ==
  in1 : Inport
  in2 : Inport  Port=2
  in3 : Inport  Port=3
  in4 : Inport  Port=4
  in5 : Inport  Port=5
  in6 : Inport  Port=6
  in7 : Inport  Port=7
  in8 : Inport  Port=8
  in9 : Inport  Port=9
  in10 : Inport  Port=10
  in11 : Inport  Port=11
  in12 : Inport  Port=12
  in13 : Inport  Port=13
  in14 : Inport  Port=14
  in15 : Inport  Port=15
  in16 : Inport  Port=16
  in17 : Inport  Port=17
  in18 : Inport  Port=18
  in19 : Inport  Port=19
  concatenate : xbsIndex_r4/Concat  num_inputs=19  dbl_ovrd=off  block_type=concat
  reinterpret{1..19} (19 alike) : xbsIndex_r4/Reinterpret  force_arith_type=on  arith_type=Unsigned  force_bin_pt=on  bin_pt=0  block_type=reinterpret
      reinterpret1 settings: infoedit="Changes signal type without altering the binary representation.   You can changed the signal between signed and unsigned, and relocate the binary point.<br><br>Hardware notes: In hardware this block costs nothing.<br><br>Example:  Suppose the input is 6 bits wide, signed, with 2 fractional bits, and the output is forced to unsigned with 0 fractional bits.  Then an input of -2.0 (1110.00 in binary 2's complement) becomes an output of 56 (111000 in binary)."
      reinterpret2 settings: infoedit="Changes signal type without altering the binary representation.   You can changed the signal between signed and unsigned, and relocate the binary point.<br><br>Hardware notes: In hardware this block costs nothing.<br><br>Example:  Suppose the input is 6 bits wide, signed, with 2 fractional bits, and the output is forced to unsigned with 0 fractional bits.  Then an input of -2.0 (1110.00 in binary 2's complement) becomes an output of 56 (111000 in binary)."
  bus_out : Outport
  wires:
  concatenate/1 -> bus_out/1
  in1/1 -> reinterpret1/1
  reinterpret1/1 -> concatenate/1
  in2/1 -> reinterpret2/1
  reinterpret2/1 -> concatenate/2
  in3/1 -> reinterpret3/1
  reinterpret3/1 -> concatenate/3
  in4/1 -> reinterpret4/1
  reinterpret4/1 -> concatenate/4
  in5/1 -> reinterpret5/1
  reinterpret5/1 -> concatenate/5
  in6/1 -> reinterpret6/1
  reinterpret6/1 -> concatenate/6
  in7/1 -> reinterpret7/1
  reinterpret7/1 -> concatenate/7
  in8/1 -> reinterpret8/1
  reinterpret8/1 -> concatenate/8
  in9/1 -> reinterpret9/1
  reinterpret9/1 -> concatenate/9
  in10/1 -> reinterpret10/1
  reinterpret10/1 -> concatenate/10
  in11/1 -> reinterpret11/1
  reinterpret11/1 -> concatenate/11
  in12/1 -> reinterpret12/1
  reinterpret12/1 -> concatenate/12
  in13/1 -> reinterpret13/1
  reinterpret13/1 -> concatenate/13
  in14/1 -> reinterpret14/1
  reinterpret14/1 -> concatenate/14
  in15/1 -> reinterpret15/1
  reinterpret15/1 -> concatenate/15
  in16/1 -> reinterpret16/1
  reinterpret16/1 -> concatenate/16
  in17/1 -> reinterpret17/1
  reinterpret17/1 -> concatenate/17
  in18/1 -> reinterpret18/1
  reinterpret18/1 -> concatenate/18
  in19/1 -> reinterpret19/1
  reinterpret19/1 -> concatenate/19

== system r2_b8a4x128f_4gbe/sys2/flags/bus_expand ==
  bus_in : Inport
  reinterpret1 : xbsIndex_r4/Reinterpret  force_arith_type=on  arith_type=Unsigned  force_bin_pt=on  bin_pt=0  block_type=reinterpret
  reinterpret2 : xbsIndex_r4/Reinterpret  force_arith_type=on  arith_type=Unsigned  force_bin_pt=on  bin_pt=0  block_type=reinterpret
  reinterpret3 : xbsIndex_r4/Reinterpret  force_arith_type=on  arith_type=Unsigned  force_bin_pt=on  bin_pt=0  block_type=reinterpret
  slice1 : xbsIndex_r4/Slice  nbits=4  boolean_output=off  mode=Upper Bit Location + Width  bit1=-16  base1=MSB of Input  bit0=0  base0=LSB of Input  dbl_ovrd=off  block_type=slice
  slice2 : xbsIndex_r4/Slice  nbits=11  boolean_output=off  mode=Upper Bit Location + Width  bit1=-5  base1=MSB of Input  bit0=0  base0=LSB of Input  dbl_ovrd=off  block_type=slice
  slice3 : xbsIndex_r4/Slice  nbits=5  boolean_output=off  mode=Upper Bit Location + Width  bit1=0  base1=MSB of Input  bit0=0  base0=LSB of Input  dbl_ovrd=off  block_type=slice
  msb_out3 : Outport
  out2 : Outport  Port=2
  lsb_out1 : Outport  Port=3
  wires:
  bus_in/1 -> slice3/1, slice2/1, slice1/1
  slice3/1 -> reinterpret3/1
  reinterpret3/1 -> msb_out3/1
  slice2/1 -> reinterpret2/1
  reinterpret2/1 -> out2/1
  slice1/1 -> reinterpret1/1
  reinterpret1/1 -> lsb_out1/1

== system r2_b8a4x128f_4gbe/sys2/flags/bus_expand1 ==
  bus_in : Inport
  reinterpret{1..4} (4 alike) : xbsIndex_r4/Reinterpret  force_arith_type=on  arith_type=Unsigned  force_bin_pt=on  bin_pt=0  block_type=reinterpret
  slice1 : xbsIndex_r4/Slice  nbits=1  boolean_output=off  mode=Upper Bit Location + Width  bit1=-3  base1=MSB of Input  bit0=0  base0=LSB of Input  dbl_ovrd=off  block_type=slice
  slice2 : xbsIndex_r4/Slice  nbits=1  boolean_output=off  mode=Upper Bit Location + Width  bit1=-2  base1=MSB of Input  bit0=0  base0=LSB of Input  dbl_ovrd=off  block_type=slice
  slice3 : xbsIndex_r4/Slice  nbits=1  boolean_output=off  mode=Upper Bit Location + Width  bit1=-1  base1=MSB of Input  bit0=0  base0=LSB of Input  dbl_ovrd=off  block_type=slice
  slice4 : xbsIndex_r4/Slice  nbits=1  boolean_output=off  mode=Upper Bit Location + Width  bit1=0  base1=MSB of Input  bit0=0  base0=LSB of Input  dbl_ovrd=off  block_type=slice
  msb_out4 : Outport
  out3 : Outport  Port=2
  out2 : Outport  Port=3
  lsb_out1 : Outport  Port=4
  wires:
  bus_in/1 -> slice4/1, slice3/1, slice2/1, slice1/1
  slice4/1 -> reinterpret4/1
  reinterpret4/1 -> msb_out4/1
  slice3/1 -> reinterpret3/1
  reinterpret3/1 -> out3/1
  slice2/1 -> reinterpret2/1
  reinterpret2/1 -> out2/1
  slice1/1 -> reinterpret1/1
  reinterpret1/1 -> lsb_out1/1
